simulink library "Contact_Forces_Lib"  (R2025b)
settings: Solver=ode45  StartTime=0.0  StopTime=10.0  RelTol=1e-3  EnableMultiTasking=on
undefined symbols (not defined in the file or in its folder): b_contact, custom_param_1, custom_param_2, Extr_Data_Ring, k_contact, l_cone, length_cylinder, length_tube, mu_kinetic, mu_static, pen_exponent, pen_full_damp_F, rad_s_cone, radius_cylinder, radius_tube, v_thr, X, Y, Z
libraries: nesl_utility x197, sm_lib x115, $bdroot x72, simulink x20, fl_lib x4
(part 11 of 12)

== system Contact_Forces_Lib/3D/Prototype/Cylinder In Ring Force/Point of Contact calc/Force Calc ==
  x : Inport
  y : Inport  Port=2
  v : Inport  Port=3
  z : Inport  Port=4
  th : Inport  Port=5
  Computing Force from nonzero penetration points : Subsystem  Commented=on
  Constant2 : Constant  Value=r_tube
  Dead Zone : DeadZone  LowerValue=-inf  UpperValue=0  ZeroCross=off
  MAX_ML : Subsystem  Commented=on
  MAX_SL : Subsystem
  Math Function : Math  Operator=square  SignedPower=on
  Math Function1 : Math  Operator=square  SignedPower=on
  Reciprocal Sqrt : Sqrt
  Sum : Sum  Inputs=|++
  Sum1 : Sum  Inputs=|+-
  Fx : Outport  VectorParamsAs1DForOutWhenUnconnected=off
  Fy : Outport  Port=2  VectorParamsAs1DForOutWhenUnconnected=off
  Fz : Outport  Port=3  VectorParamsAs1DForOutWhenUnconnected=off
  pc : Outport  Port=4  VectorParamsAs1DForOutWhenUnconnected=off
  maxpen : Outport  Port=5  VectorParamsAs1DForOutWhenUnconnected=off
  wires:
  y/1 -> MAX_SL/1(Y), Math Function1/1
  x/1 -> MAX_SL/2(X), Math Function/1
  Sum/1 -> Reciprocal Sqrt/1
  Reciprocal Sqrt/1 -> Sum1/1
  Constant2/1 -> Sum1/2
  Sum1/1 -> Dead Zone/1
  MAX_SL/1(Fx) -> Fx/1
  MAX_SL/2(Fy) -> Fy/1
  Dead Zone/1 -> MAX_SL/3(Pen)
  Math Function1/1 -> Sum/1
  Math Function/1 -> Sum/2
  v/1 -> MAX_SL/4(v)
  th/1 -> MAX_SL/5(th)
  z/1 -> MAX_SL/6(z)
  MAX_SL/4(pc) -> pc/1
  MAX_SL/3(Fz) -> Fz/1
  MAX_SL/5(maxpen) -> maxpen/1

== system Contact_Forces_Lib/3D/Prototype/Cylinder In Ring Force/Point of Contact calc/x calc ==
  note: Xb = r11*r*cos(th) + r12*r*sin(th) +r13*z + Xc;
  note: Find x coordinate in tube frame for cylinder point that is in the plane of the end of the tube
  r11 : Inport
  r12 : Inport  Port=2
  r13 : Inport  Port=3
  xc : Inport  Port=4
  th : Inport  Port=5
  z : Inport  Port=6
  Gain : Gain  Gain=r_cyl
  Gain1 : Gain  Gain=r_cyl
  Product : Product
  Product1 : Product
  Product2 : Product
  Sum : Sum  Inputs=|++++
  Trigonometric Function : Trigonometry  Operator=cos
  Trigonometric Function1 : Trigonometry
  x : Outport  VectorParamsAs1DForOutWhenUnconnected=off
  wires:
  th/1 -> Trigonometric Function/1, Trigonometric Function1/1
  Sum/1 -> x/1
  Product/1 -> Gain/1
  Gain1/1 -> Sum/3
  Trigonometric Function/1 -> Product/2
  Trigonometric Function1/1 -> Product1/2
  Gain/1 -> Sum/2
  Product1/1 -> Gain1/1
  r11/1 -> Product/1
  r12/1 -> Product1/1
  xc/1 -> Sum/1
  r13/1 -> Product2/1
  z/1 -> Product2/2
  Product2/1 -> Sum/4

== system Contact_Forces_Lib/3D/Prototype/Cylinder In Ring Force/Point of Contact calc/y calc ==
  note: Yb = r21*r*cos(th) + r22*r*sin(th) +r23*z + Yc;
  note: Find y coordinate in tube frame for cylinder point that is in the plane of the end of the tube
  r21 : Inport
  r22 : Inport  Port=2
  r23 : Inport  Port=3
  yc : Inport  Port=4
  th : Inport  Port=5
  z : Inport  Port=6
  Gain : Gain  Gain=r_cyl
  Gain1 : Gain  Gain=r_cyl
  Product : Product
  Product1 : Product
  Product2 : Product
  Sum : Sum  Inputs=|++++
  Trigonometric Function : Trigonometry  Operator=cos
  Trigonometric Function1 : Trigonometry
  y : Outport  VectorParamsAs1DForOutWhenUnconnected=off
  wires:
  Product2/1 -> Sum/4
  z/1 -> Product2/2
  r23/1 -> Product2/1
  yc/1 -> Sum/1
  r22/1 -> Product1/1
  r21/1 -> Product/1
  Product1/1 -> Gain1/1
  Gain/1 -> Sum/2
  Trigonometric Function1/1 -> Product1/2
  Trigonometric Function/1 -> Product/2
  Gain1/1 -> Sum/3
  Product/1 -> Gain/1
  Sum/1 -> y/1
  th/1 -> Trigonometric Function1/1, Trigonometric Function/1

== system Contact_Forces_Lib/3D/Prototype/Cylinder In Ring Force/Point of Contact calc/z calc ==
  note: Find z coordinate in cylinder frame for cylinder point that is in the plane of the end of the tube
  note: z = (L/2 - r31*r*cos(th) - r32*r*sin(th) - Zc)/r33;
  r31 : Inport
  r32 : Inport  Port=2
  r33 : Inport  Port=3
  zc : Inport  Port=4
  th : Inport  Port=5
  Constant : Constant  Value=l_tube/2
  Divide : Product  Inputs=*/
  Gain : Gain  Gain=r_cyl
  Gain1 : Gain  Gain=r_cyl
  Product : Product
  Product1 : Product
  Sum : Sum  Inputs=|---+
  Trigonometric Function : Trigonometry  Operator=cos
  Trigonometric Function1 : Trigonometry
  z : Outport  VectorParamsAs1DForOutWhenUnconnected=off
  wires:
  r32/1 -> Product1/1
  r31/1 -> Product/1
  Product1/1 -> Gain1/1
  Gain/1 -> Sum/2
  Trigonometric Function1/1 -> Product1/2
  Trigonometric Function/1 -> Product/2
  Gain1/1 -> Sum/3
  Product/1 -> Gain/1
  r33/1 -> Divide/2
  Constant/1 -> Sum/4
  Sum/1 -> Divide/1
  Divide/1 -> z/1
  zc/1 -> Sum/1
  th/1 -> Trigonometric Function1/1, Trigonometric Function/1

== system Contact_Forces_Lib/3D/Sphere in Sphere Force/Ff/Check w or v non zero/Else ==
  Action Port : ActionPort
  vabs_zero : Constant  Value=0  SampleTime=0
  vuvect_zero : Constant  Value=[0 0 0]  SampleTime=0
  vabs : Outport  InitialOutput=0  VectorParamsAs1DForOutWhenUnconnected=off
  vuvect : Outport  Port=2  InitialOutput=0  VectorParamsAs1DForOutWhenUnconnected=off
  wires:
  vabs_zero/1 -> vabs/1
  vuvect_zero/1 -> vuvect/1

== system Contact_Forces_Lib/3D/Sphere in Sphere Force/Ff/Check w or v non zero/mag v ==
  vect : Inport
  Add2 : Sum  Inputs=+++
  Demux : Demux  Outputs=3
  Math Function : Math  Operator=square  SignedPower=on
  Math Function1 : Math  Operator=square  SignedPower=on
  Math Function2 : Math  Operator=square  SignedPower=on
  Sqrt : Sqrt
  mag : Outport  VectorParamsAs1DForOutWhenUnconnected=off
  wires:
  Math Function2/1 -> Add2/3
  Demux/3 -> Math Function2/1
  Sqrt/1 -> mag/1
  Math Function1/1 -> Add2/2
  Math Function/1 -> Add2/1
  Add2/1 -> Sqrt/1
  vect/1 -> Demux/1
  Demux/1 -> Math Function/1
  Demux/2 -> Math Function1/1

== system Contact_Forces_Lib/3D/Sphere in Sphere Force/Ff/Check w or v non zero/mag w ==
  vect : Inport
  Add : Sum  Inputs=+++
  Demux : Demux  Outputs=3
  Math Function : Math  Operator=square  SignedPower=on
  Math Function1 : Math  Operator=square  SignedPower=on
  Math Function2 : Math  Operator=square  SignedPower=on
  Sqrt : Sqrt
  mag : Outport  VectorParamsAs1DForOutWhenUnconnected=off
  wires:
  Demux/2 -> Math Function1/1
  Demux/1 -> Math Function/1
  vect/1 -> Demux/1
  Add/1 -> Sqrt/1
  Math Function/1 -> Add/1
  Math Function1/1 -> Add/2
  Sqrt/1 -> mag/1
  Demux/3 -> Math Function2/1
  Math Function2/1 -> Add/3

== system Contact_Forces_Lib/3D/Sphere in Sphere Force/Ff/SlipVel/If Action Subsystem ==
  In1 : Inport
  In2 : Inport  Port=2
  Action Port : ActionPort
  Divide : Product  Inputs=/*
  Out1 : Outport  VectorParamsAs1DForOutWhenUnconnected=off
  wires:
  Divide/1 -> Out1/1
  In2/1 -> Divide/2
  In1/1 -> Divide/1

== system Contact_Forces_Lib/3D/Sphere in Sphere Force/Ff/SlipVel/mag ==
  vect : Inport
  Add2 : Sum  Inputs=+++
  Demux : Demux  Outputs=3
  Math Function : Math  Operator=square  SignedPower=on
  Math Function1 : Math  Operator=square  SignedPower=on
  Math Function2 : Math  Operator=square  SignedPower=on
  Sqrt : Sqrt
  mag : Outport  VectorParamsAs1DForOutWhenUnconnected=off
  wires:
  Math Function2/1 -> Add2/3
  Demux/3 -> Math Function2/1
  Sqrt/1 -> mag/1
  Math Function1/1 -> Add2/2
  Math Function/1 -> Add2/1
  Add2/1 -> Sqrt/1
  vect/1 -> Demux/1
  Demux/1 -> Math Function/1
  Demux/2 -> Math Function1/1

== system Contact_Forces_Lib/3D/Sphere to Cone Force/Forces/Ff/Relative vel at CP ==
  note: Calculate relative velocity at contact point between sphere and tube. Two components: about ring and along tube axis. Use magnitude to calculate friction force, atan2 retains relative magnitude and direction between the components.
  InOut : Inport
  rad : Inport  Port=2
  vrad : Inport  Port=3
  Pen : Inport  Port=4
  vazm : Inport  Port=5
  vazmx : Inport  Port=6
  vazmy : Inport  Port=7
  wzf : Inport  Port=8
  vzf : Inport  Port=9
  wxf : Inport  Port=10
  wyf : Inport  Port=11
  azm : Inport  Port=12
  Calculate vRelFace : Subsystem
  Calculate vRelRing : Subsystem
  Follower Radius : Constant  Value=radius_sphere
  Math Function : Math  Operator=square  SignedPower=on
  Math Function1 : Math  Operator=square  SignedPower=on
  Midpt Pen : Gain  Gain=0.5
  Product1 : Product
  Sqrt : Sqrt
  Sum1 : Sum  Inputs=+-
  Sum3 : Sum  Inputs=|++
  Trigonometric Function : Trigonometry  Operator=atan2
  vRelAbs : Outport  VectorParamsAs1DForOutWhenUnconnected=off
  rSphtoCP : Outport  Port=2  VectorParamsAs1DForOutWhenUnconnected=off
  rConAxtoCP : Outport  Port=3  VectorParamsAs1DForOutWhenUnconnected=off
  alpha : Outport  Port=4  VectorParamsAs1DForOutWhenUnconnected=off
  wires:
  vrad/1 -> Calculate vRelFace/6(vrad)
  vazmy/1 -> Calculate vRelRing/6(vazmy)
  vazmx/1 -> Calculate vRelRing/5(vazmx)
  Product1/1 -> Calculate vRelRing/1(rSphtoCP sign), Calculate vRelFace/1(rSphtoCP sign)
  Sum1/1 -> Product1/1, rSphtoCP/1  "rSphtoCP"
  InOut/1 -> Product1/2  "InOut"
  Trigonometric Function/1 -> alpha/1  "alpha"
  Sqrt/1 -> vRelAbs/1
  Sum3/1 -> Sqrt/1
  Math Function/1 -> Sum3/1
  Math Function1/1 -> Sum3/2
  Follower Radius/1 -> Sum1/1
  Pen/1 -> Midpt Pen/1
  Midpt Pen/1 -> Sum1/2
  Calculate vRelFace/1(vRelFace) -> Math Function1/1, Trigonometric Function/1  "vRelFace"
  wxf/1 -> Calculate vRelFace/3(wxf), Calculate vRelRing/8(wxf)
  vzf/1 -> Calculate vRelFace/5(vzf)
  azm/1 -> Calculate vRelFace/2(azm), Calculate vRelRing/7(azm)
  wyf/1 -> Calculate vRelRing/9(wyf), Calculate vRelFace/4(wyf)
  Calculate vRelRing/2(vRelRing) -> Math Function/1, Trigonometric Function/2  "vRelRing"
  rad/1 -> Calculate vRelRing/2(rad)
  vazm/1 -> Calculate vRelRing/3(vazm)
  wzf/1 -> Calculate vRelRing/4(wzf)
  Calculate vRelRing/1(rConAxtoCP) -> rConAxtoCP/1

== system Contact_Forces_Lib/3D/Sphere to Cone Force/Forces/Ff/Resolve Ff ==
  note: Resolve Friction Force in
      | Sphere F reference frame
  note: Resolve Friction Force in
      | Cone B reference frame
  InOut : Inport
  Ff : Inport  Port=2
  R : Inport  Port=3
  z : Inport  Port=4
  rSphtoCP : Inport  Port=5
  rConAxtoCP : Inport  Port=6
  alpha : Inport  Port=7
  azm : Inport  Port=8
  Ff in ConB : Subsystem
  Ff in SphF : Subsystem
  FxSphF : Outport  VectorParamsAs1DForOutWhenUnconnected=off
  FySphF : Outport  Port=2  VectorParamsAs1DForOutWhenUnconnected=off
  FzSphF : Outport  Port=3  VectorParamsAs1DForOutWhenUnconnected=off
  TSphF : Outport  Port=4  VectorParamsAs1DForOutWhenUnconnected=off
  FxConB : Outport  Port=5  VectorParamsAs1DForOutWhenUnconnected=off
  FyConB : Outport  Port=6  VectorParamsAs1DForOutWhenUnconnected=off
  FzConB : Outport  Port=7  VectorParamsAs1DForOutWhenUnconnected=off
  TConB : Outport  Port=8  VectorParamsAs1DForOutWhenUnconnected=off
  wires:
  Ff in SphF/4(TSphF) -> TSphF/1
  Ff in ConB/4(TSphF_B) -> Ff in SphF/4(TSphF_B)
  Ff in ConB/5(TConB) -> TConB/1
  alpha/1 -> Ff in ConB/4(alpha)
  Ff in ConB/3(FzConB) -> FzConB/1, Ff in SphF/3(FzConB)
  Ff in SphF/3(FzSphF) -> FzSphF/1
  R/1 -> Ff in SphF/5(R)
  azm/1 -> Ff in ConB/3(azm)
  Ff in SphF/2(FxSphF) -> FxSphF/1
  Ff in ConB/2(FyConB) -> Ff in SphF/2(FyConB), FyConB/1
  Ff in ConB/1(FxConB) -> FxConB/1, Ff in SphF/1(FxConB)
  Ff in SphF/1(FySphF) -> FySphF/1
  Ff/1 -> Ff in ConB/2(Ff)
  rConAxtoCP/1 -> Ff in ConB/6(rConAxtoCP)
  rSphtoCP/1 -> Ff in ConB/5(rSphtoCP)
  z/1 -> Ff in ConB/7(z)
  InOut/1 -> Ff in ConB/1(InOut)

== system Contact_Forces_Lib/3D/Sphere to Cone Force/Forces/Fn/Equiv Torques ==
  azm : Inport
  FxConB : Inport  Port=2
  FyConB : Inport  Port=3
  FzConB : Inport  Port=4
  rad : Inport  Port=5
  z : Inport  Port=6
  Constant : Constant  Value=radius_sphere*sinConeTh
  Constant1 : Constant  Value=radius_sphere*cosConeTh
  Product : Product  Inputs=3
  Product1 : Product
  Product2 : Product  Inputs=3
  Product3 : Product
  Sum : Sum
  Sum1 : Sum  Inputs=+-
  Sum2 : Sum
  Sum3 : Sum  Inputs=+-
  sin : Trigonometry
  sin1 : Trigonometry  Operator=cos
  TxConB : Outport  VectorParamsAs1DForOutWhenUnconnected=off
  TyConB : Outport  Port=2  VectorParamsAs1DForOutWhenUnconnected=off
  wires:
  sin1/1 -> Product2/2
  sin/1 -> Product/2
  Sum/1 -> Product/3, Product2/3
  Sum3/1 -> TyConB/1
  Sum1/1 -> TxConB/1
  rad/1 -> Sum/1
  Product3/1 -> Sum3/1
  Product/1 -> Sum1/1
  Constant1/1 -> Sum2/2
  Sum2/1 -> Product3/2, Product1/2
  Constant/1 -> Sum/2
  z/1 -> Sum2/1
  Product1/1 -> Sum1/2
  Product2/1 -> Sum3/2
  azm/1 -> sin/1, sin1/1
  FxConB/1 -> Product3/1
  FzConB/1 -> Product/1, Product2/1
  FyConB/1 -> Product1/1

== system Contact_Forces_Lib/3D/Sphere to Cone Force/Forces/Fn/Fn in SphF ==
  R : Inport
  FxConB : Inport  Port=2
  FyConB : Inport  Port=3
  FzConB : Inport  Port=4
  Demux : Demux  Outputs=3
  Divide3 : Product  Inputs=/*  Multiplication=Matrix(*)
  Gain : Gain  Gain=-1
  Mux1 : Mux  Inputs=3
  FySphF : Outport  VectorParamsAs1DForOutWhenUnconnected=off
  FxSphF : Outport  Port=2  VectorParamsAs1DForOutWhenUnconnected=off
  FzSphF : Outport  Port=3  VectorParamsAs1DForOutWhenUnconnected=off
  wires:
  FzConB/1 -> Mux1/3
  Gain/1 -> Demux/1
  R/1 -> Divide3/1
  Demux/1 -> FxSphF/1
  Demux/2 -> FySphF/1
  Demux/3 -> FzSphF/1
  FxConB/1 -> Mux1/1
  FyConB/1 -> Mux1/2
  Mux1/1 -> Divide3/2
  Divide3/1 -> Gain/1

== system Contact_Forces_Lib/3D/Sphere to Cone Force/Forces/Fn/Fn in TubB ==
  Fn : Inport
  azm : Inport  Port=2
  Divide1 : Product  Inputs=**
  Divide2 : Product  Inputs=**
  Gain : Gain  Gain=sinConeTh
  Gain1 : Gain  Gain=sinConeTh
  cos : Trigonometry  Operator=cos
  sin : Trigonometry
  FxConB : Outport  VectorParamsAs1DForOutWhenUnconnected=off
  FyConB : Outport  Port=2  VectorParamsAs1DForOutWhenUnconnected=off
  FzConB : Outport  Port=3  VectorParamsAs1DForOutWhenUnconnected=off
  wires:
  Gain1/1 -> FzConB/1
  Gain/1 -> Divide1/1, Divide2/1
  Fn/1 -> Gain/1, Gain1/1
  azm/1 -> cos/1, sin/1
  sin/1 -> Divide2/2
  cos/1 -> Divide1/2
  Divide1/1 -> FxConB/1
  Divide2/1 -> FyConB/1

== system Contact_Forces_Lib/3D/Sphere to Cone Force/Sensing/rad_azm_cal/rad_0 ==
  Action Port : ActionPort
  Zeros : Constant  Value=[0 0 0 0]  SampleTime=0
  F : Outport  InitialOutput=[0]  VectorParamsAs1DForOutWhenUnconnected=off
  wires:
  Zeros/1 -> F/1

== system Contact_Forces_Lib/3D/Sphere to Cone Force/Sensing/rad_azm_cal/rad_azm_cal ==
  note: vazm = (x*vy - y*vx)/(x^2+y^2)
  note: vrad = (x*vx + y*vy)/z
  note: azm = atan2(y, x)
  note: rad = sqrt(x^2+y^2)
  x : Inport
  y : Inport  Port=2
  vx : Inport  Port=3
  vy : Inport  Port=4
  Action Port : ActionPort
  Add : Sum
  Add1 : Sum  Inputs=+-
  Divide : Product  Inputs=*/
  Divide1 : Product  Inputs=*/
  Math Function : Math  Operator=square  SignedPower=on
  Math Function1 : Math  Operator=square  SignedPower=on
  Mux : Mux
  Product{,1..3} (4 alike) : Product
  Sqrt : Sqrt
  Sum : Sum
  Trigonometric Function : Trigonometry  Operator=atan2
  F : Outport  VectorParamsAs1DForOutWhenUnconnected=off
  wires:
  Math Function1/1 -> Sum/2
  Math Function/1 -> Sum/1
  Sum/1 -> Divide1/2, Sqrt/1
  Trigonometric Function/1 -> Mux/2  "azm"
  x/1 -> Trigonometric Function/2, Product/1, Product2/1, Math Function/1
  y/1 -> Trigonometric Function/1, Product1/1, Product3/1, Math Function1/1
  vx/1 -> Product3/2, Product/2
  vy/1 -> Product2/2, Product1/2
  Product/1 -> Add/1
  Product1/1 -> Add/2
  Add/1 -> Divide/1
  Sqrt/1 -> Mux/1, Divide/2  "rad"
  Divide/1 -> Mux/3  "vrad"
  Product2/1 -> Add1/1
  Product3/1 -> Add1/2
  Add1/1 -> Divide1/1
  Divide1/1 -> Mux/4  "vazm"
  Mux/1 -> F/1

== system Contact_Forces_Lib/3D/Sphere to Cone Force/Sensing/rad_azm_cal/vazmx_0 ==
  Action Port : ActionPort
  Zeros : Constant  Value=0  SampleTime=0
  F : Outport  InitialOutput=[0]  VectorParamsAs1DForOutWhenUnconnected=off
  wires:
  Zeros/1 -> F/1

== system Contact_Forces_Lib/3D/Sphere to Cone Force/Sensing/rad_azm_cal/vazmx_cal ==
  note: vazmx = (y*vz - z*vy)/(y^2+z^2)
  y : Inport
  z : Inport  Port=2
  vy : Inport  Port=3
  vz : Inport  Port=4
  Action Port : ActionPort
  Add2 : Sum  Inputs=+-
  Divide2 : Product  Inputs=*/
  Math Function1 : Math  Operator=square  SignedPower=on
  Math Function2 : Math  Operator=square  SignedPower=on
  Product4 : Product
  Product5 : Product
  Sum1 : Sum
  vazmx : Outport  VectorParamsAs1DForOutWhenUnconnected=off
  wires:
  Product4/1 -> Add2/1
  Product5/1 -> Add2/2
  Add2/1 -> Divide2/1
  vy/1 -> Product5/2
  y/1 -> Math Function1/1, Product4/1
  Math Function1/1 -> Sum1/1
  z/1 -> Product5/1, Math Function2/1
  Math Function2/1 -> Sum1/2
  Sum1/1 -> Divide2/2
  vz/1 -> Product4/2
  Divide2/1 -> vazmx/1  "vazmx"

== system Contact_Forces_Lib/3D/Sphere to Cone Force/Sensing/rad_azm_cal/vazmy_0 ==
  Action Port : ActionPort
  Zeros : Constant  Value=0  SampleTime=0
  F : Outport  InitialOutput=[0]  VectorParamsAs1DForOutWhenUnconnected=off
  wires:
  Zeros/1 -> F/1

== system Contact_Forces_Lib/3D/Sphere to Cone Force/Sensing/rad_azm_cal/vazmy_cal ==
  note: vazmy = (z*vx - x*vz)/(z^2+x^2)
  x : Inport
  z : Inport  Port=2
  vx : Inport  Port=3
  vz : Inport  Port=4
  Action Port : ActionPort
  Add3 : Sum  Inputs=+-
  Divide3 : Product  Inputs=*/
  Math Function : Math  Operator=square  SignedPower=on
  Math Function2 : Math  Operator=square  SignedPower=on
  Product6 : Product
  Product7 : Product
  Sum2 : Sum
  vazmy : Outport  VectorParamsAs1DForOutWhenUnconnected=off
  wires:
  vx/1 -> Product6/2
  x/1 -> Math Function/1, Product7/1
  Math Function/1 -> Sum2/1
  Add3/1 -> Divide3/1
  Product7/1 -> Add3/2
  Product6/1 -> Add3/1
  z/1 -> Product6/1, Math Function2/1
  Math Function2/1 -> Sum2/2
  Sum2/1 -> Divide3/2
  vz/1 -> Product7/2
  Divide3/1 -> vazmy/1  "vazmy"

== system Contact_Forces_Lib/3D/Sphere to Plane Force/Forces/Ff/SlipVel ==
  wx : Inport
  wy : Inport  Port=2
  vx : Inport  Port=3
  vy : Inport  Port=4
  Fx1 : Constant  Value=sphere_rad
  Math Function : Math  Operator=square  SignedPower=on
  Math Function1 : Math  Operator=square  SignedPower=on
  Product3 : Product
  Product4 : Product
  Sqrt : Sqrt
  Sum1 : Sum  Inputs=|++
  Sum2 : Sum  Inputs=|-+
  Sum3 : Sum  Inputs=|++
  Trigonometric Function : Trigonometry  Operator=atan2
  vabs : Outport  VectorParamsAs1DForOutWhenUnconnected=off
  alpha : Outport  Port=2  VectorParamsAs1DForOutWhenUnconnected=off
  wires:
  Sum2/1 -> Math Function1/1, Trigonometric Function/2  "slipx"
  Sum1/1 -> Math Function/1, Trigonometric Function/1  "slipy"
  Math Function1/1 -> Sum3/2
  Math Function/1 -> Sum3/1
  Sum3/1 -> Sqrt/1
  Sqrt/1 -> vabs/1
  Trigonometric Function/1 -> alpha/1
  Product4/1 -> Sum2/1
  vy/1 -> Sum1/2
  Fx1/1 -> Product4/1, Product3/2
  vx/1 -> Sum2/2
  wy/1 -> Product4/2
  Product3/1 -> Sum1/1
  wx/1 -> Product3/1

== system Contact_Forces_Lib/3D/Sphere to Plane Force Enabled/Forces/Ff/SlipVel ==
  wx : Inport
  wy : Inport  Port=2
  vx : Inport  Port=3
  vy : Inport  Port=4
  Fx1 : Constant  Value=sphere_rad
  Math Function : Math  Operator=square  SignedPower=on
  Math Function1 : Math  Operator=square  SignedPower=on
  Product3 : Product
  Product4 : Product
  Sqrt : Sqrt
  Sum1 : Sum  Inputs=|++
  Sum2 : Sum  Inputs=|-+
  Sum3 : Sum  Inputs=|++
  Trigonometric Function : Trigonometry  Operator=atan2
  vabs : Outport  VectorParamsAs1DForOutWhenUnconnected=off
  alpha : Outport  Port=2  VectorParamsAs1DForOutWhenUnconnected=off
  wires:
  wx/1 -> Product3/1
  Product3/1 -> Sum1/1
  wy/1 -> Product4/2
  vx/1 -> Sum2/2
  Fx1/1 -> Product3/2, Product4/1
  vy/1 -> Sum1/2
  Product4/1 -> Sum2/1
  Trigonometric Function/1 -> alpha/1
  Sqrt/1 -> vabs/1
  Sum3/1 -> Sqrt/1
  Math Function/1 -> Sum3/1
  Math Function1/1 -> Sum3/2
  Sum1/1 -> Trigonometric Function/1, Math Function/1  "slipy"
  Sum2/1 -> Trigonometric Function/2, Math Function1/1  "slipx"

== system Contact_Forces_Lib/3D/Sphere to Sphere Force/Ff/Check w or v non zero/Else ==
  Action Port : ActionPort
  Constant : Constant  Value=0  SampleTime=0
  Constant1 : Constant  Value=[0 0 0]  SampleTime=0
  vabs : Outport  InitialOutput=0  VectorParamsAs1DForOutWhenUnconnected=off
  vuvect : Outport  Port=2  InitialOutput=0  VectorParamsAs1DForOutWhenUnconnected=off
  wires:
  Constant1/1 -> vuvect/1
  Constant/1 -> vabs/1

== system Contact_Forces_Lib/3D/Sphere to Sphere Force/Ff/Check w or v non zero/mag v ==
  vect : Inport
  Add2 : Sum  Inputs=+++
  Demux : Demux  Outputs=3
  Math Function : Math  Operator=square  SignedPower=on
  Math Function1 : Math  Operator=square  SignedPower=on
  Math Function2 : Math  Operator=square  SignedPower=on
  Sqrt : Sqrt
  mag : Outport  VectorParamsAs1DForOutWhenUnconnected=off
  wires:
  Demux/2 -> Math Function1/1
  Demux/1 -> Math Function/1
  vect/1 -> Demux/1
  Add2/1 -> Sqrt/1
  Math Function/1 -> Add2/1
  Math Function1/1 -> Add2/2
  Sqrt/1 -> mag/1
  Demux/3 -> Math Function2/1
  Math Function2/1 -> Add2/3

== system Contact_Forces_Lib/3D/Sphere to Sphere Force/Ff/Check w or v non zero/mag w ==
  vect : Inport
  Add : Sum  Inputs=+++
  Demux : Demux  Outputs=3
  Math Function : Math  Operator=square  SignedPower=on
  Math Function1 : Math  Operator=square  SignedPower=on
  Math Function2 : Math  Operator=square  SignedPower=on
  Sqrt : Sqrt
  mag : Outport  VectorParamsAs1DForOutWhenUnconnected=off
  wires:
  Math Function2/1 -> Add/3
  Demux/3 -> Math Function2/1
  Sqrt/1 -> mag/1
  Math Function1/1 -> Add/2
  Math Function/1 -> Add/1
  Add/1 -> Sqrt/1
  vect/1 -> Demux/1
  Demux/1 -> Math Function/1
  Demux/2 -> Math Function1/1

== system Contact_Forces_Lib/3D/Sphere to Sphere Force/Ff/SlipVel/If Action Subsystem ==
  In1 : Inport
  In2 : Inport  Port=2
  Action Port : ActionPort
  Divide : Product  Inputs=/*
  Out1 : Outport  VectorParamsAs1DForOutWhenUnconnected=off
  wires:
  In1/1 -> Divide/1
  In2/1 -> Divide/2
  Divide/1 -> Out1/1

== system Contact_Forces_Lib/3D/Sphere to Sphere Force/Ff/SlipVel/mag ==
  vect : Inport
  Add2 : Sum  Inputs=+++
  Demux : Demux  Outputs=3
  Math Function : Math  Operator=square  SignedPower=on
  Math Function1 : Math  Operator=square  SignedPower=on
  Math Function2 : Math  Operator=square  SignedPower=on
  Sqrt : Sqrt
  mag : Outport  VectorParamsAs1DForOutWhenUnconnected=off
  wires:
  Demux/2 -> Math Function1/1
  Demux/1 -> Math Function/1
  vect/1 -> Demux/1
  Add2/1 -> Sqrt/1
  Math Function/1 -> Add2/1
  Math Function1/1 -> Add2/2
  Sqrt/1 -> mag/1
  Demux/3 -> Math Function2/1
  Math Function2/1 -> Add2/3

== system Contact_Forces_Lib/3D/Sphere to Tube Force/Forces/Ff/Relative vel at CP ==
  note: Calculate relative velocity at contact point between sphere and tube. Two components: about ring and along tube axis. Use magnitude to calculate friction force, atan2 retains relative magnitude and direction between the components.
  Fn : Inport
  rad : Inport  Port=2
  Pen : Inport  Port=3
  vazm : Inport  Port=4
  wzf : Inport  Port=5
  vzf : Inport  Port=6
  wxf : Inport  Port=7
  wyf : Inport  Port=8
  azm : Inport  Port=9
  Calculate vRelAxis : Subsystem
  Calculate vRelRing : Subsystem
  Follower Radius : Constant  Value=radius_sphere
  Math Function : Math  Operator=square  SignedPower=on
  Math Function1 : Math  Operator=square  SignedPower=on
  Midpt Pen : Gain  Gain=0.5
  Product1 : Product
  Sign : Signum  ZeroCross=off
  Sqrt : Sqrt
  Sum1 : Sum  Inputs=+-
  Sum3 : Sum  Inputs=|++
  Trigonometric Function : Trigonometry  Operator=atan2
  vRelAbs : Outport  VectorParamsAs1DForOutWhenUnconnected=off
  rSphtoCP : Outport  Port=2  VectorParamsAs1DForOutWhenUnconnected=off
  rCyltoCP : Outport  Port=3  VectorParamsAs1DForOutWhenUnconnected=off
  alpha : Outport  Port=4  VectorParamsAs1DForOutWhenUnconnected=off
  wires:
  Calculate vRelRing/1(rCyltoCP) -> rCyltoCP/1
  wzf/1 -> Calculate vRelRing/3(wzf)
  vazm/1 -> Calculate vRelRing/2(vazm)
  rad/1 -> Calculate vRelRing/1(rad)
  Calculate vRelRing/2(vRelRing) -> Math Function/1, Trigonometric Function/2  "vRelRing"
  wyf/1 -> Calculate vRelAxis/5(wyf)
  azm/1 -> Calculate vRelAxis/4(azm)
  vzf/1 -> Calculate vRelAxis/3(vzf)
  wxf/1 -> Calculate vRelAxis/2(wxf)
  Calculate vRelAxis/1(vRelAxis) -> Trigonometric Function/1, Math Function1/1  "vRelAxis"
  Midpt Pen/1 -> Sum1/2
  Fn/1 -> Sign/1
  Pen/1 -> Midpt Pen/1
  Follower Radius/1 -> Sum1/1
  Math Function1/1 -> Sum3/2
  Math Function/1 -> Sum3/1
  Sum3/1 -> Sqrt/1
  Sqrt/1 -> vRelAbs/1
  Trigonometric Function/1 -> alpha/1  "alpha"
  Sign/1 -> Product1/2  "InOut"
  Sum1/1 -> Product1/1, rSphtoCP/1  "rSphtoCP"
  Product1/1 -> Calculate vRelAxis/1(rSphtoCP sign), Calculate vRelRing/4(rSphtoCP sign)

== system Contact_Forces_Lib/3D/Sphere to Tube Force/Forces/Ff/Resolve Ff ==
  note: Resolve Friction Force in
      | Tube B reference frame
  note: Resolve Friction Force in
      | Sphere F reference frame
  InOut : Inport
  Ff : Inport  Port=2
  rSphtoCP : Inport  Port=3
  rCyltoCP : Inport  Port=4
  alpha : Inport  Port=5
  z : Inport  Port=6
  R : Inport  Port=7
  azm : Inport  Port=8
  Ff in SphF : Subsystem
  Ff in TubB : Subsystem
  FxSphF : Outport  VectorParamsAs1DForOutWhenUnconnected=off
  FySphF : Outport  Port=2  VectorParamsAs1DForOutWhenUnconnected=off
  FzSphF : Outport  Port=3  VectorParamsAs1DForOutWhenUnconnected=off
  TSphF : Outport  Port=4  VectorParamsAs1DForOutWhenUnconnected=off
  FxSphB : Outport  Port=5  VectorParamsAs1DForOutWhenUnconnected=off
  FyTubB : Outport  Port=6  VectorParamsAs1DForOutWhenUnconnected=off
  FzTubB : Outport  Port=7  VectorParamsAs1DForOutWhenUnconnected=off
  TTubB : Outport  Port=8  VectorParamsAs1DForOutWhenUnconnected=off
  wires:
  InOut/1 -> Ff in TubB/1(InOut)
  z/1 -> Ff in TubB/7(z)
  rSphtoCP/1 -> Ff in TubB/5(rSphtoCP)
  rCyltoCP/1 -> Ff in TubB/6(rCyltoCP)
  Ff/1 -> Ff in TubB/2(Ff)
  Ff in SphF/1(FySphF) -> FySphF/1
  Ff in TubB/1(FxTubB) -> Ff in SphF/1(FxTubB), FxSphB/1
  Ff in TubB/2(FyTubB) -> FyTubB/1, Ff in SphF/2(FyTubB)
  Ff in SphF/2(FxSphF) -> FxSphF/1
  azm/1 -> Ff in TubB/3(azm)
  R/1 -> Ff in SphF/5(R)
  Ff in SphF/3(FzSphF) -> FzSphF/1
  Ff in TubB/3(FzTubB) -> Ff in SphF/3(FzTubB), FzTubB/1
  alpha/1 -> Ff in TubB/4(alpha)
  Ff in TubB/5(TTubB) -> TTubB/1
  Ff in TubB/4(TSphF_B) -> Ff in SphF/4(TSphF_B)
  Ff in SphF/4(TSphF) -> TSphF/1

== system Contact_Forces_Lib/3D/Sphere to Tube Force/Forces/Fn/Fn in SphF ==
  R : Inport
  FxTubB : Inport  Port=2
  FyTubB : Inport  Port=3
  Constant : Constant  Value=0
  Demux : Demux  Outputs=3
  Divide3 : Product  Inputs=/*  Multiplication=Matrix(*)
  Gain : Gain  Gain=-1
  Mux1 : Mux  Inputs=3
  FySphF : Outport  VectorParamsAs1DForOutWhenUnconnected=off
  FxSphF : Outport  Port=2  VectorParamsAs1DForOutWhenUnconnected=off
  FzSphF : Outport  Port=3  VectorParamsAs1DForOutWhenUnconnected=off
  wires:
  Divide3/1 -> Gain/1
  Mux1/1 -> Divide3/2
  FyTubB/1 -> Mux1/2
  FxTubB/1 -> Mux1/1
  Demux/3 -> FzSphF/1
  Demux/2 -> FySphF/1
  Demux/1 -> FxSphF/1
  Constant/1 -> Mux1/3
  R/1 -> Divide3/1
  Gain/1 -> Demux/1

== system Contact_Forces_Lib/3D/Sphere to Tube Force/Forces/Fn/Fn in TubB ==
  Fn : Inport
  azm : Inport  Port=2
  Divide1 : Product  Inputs=**
  Divide2 : Product  Inputs=**
  cos : Trigonometry  Operator=cos
  sin : Trigonometry
  FxTubB : Outport  VectorParamsAs1DForOutWhenUnconnected=off
  FyTubB : Outport  Port=2  VectorParamsAs1DForOutWhenUnconnected=off
  wires:
  Divide2/1 -> FyTubB/1
  Divide1/1 -> FxTubB/1
  cos/1 -> Divide1/2
  sin/1 -> Divide2/2
  azm/1 -> sin/1, cos/1
  Fn/1 -> Divide2/1, Divide1/1

== system Contact_Forces_Lib/3D/Sphere to Tube Force/Sensing/rad_azm_cal/rad_0 ==
  Action Port : ActionPort
  Zeros : Constant  Value=[0 0 0 0]  SampleTime=0
  F : Outport  InitialOutput=[0]  VectorParamsAs1DForOutWhenUnconnected=off
  wires:
  Zeros/1 -> F/1

== system Contact_Forces_Lib/3D/Sphere to Tube Force/Sensing/rad_azm_cal/rad_azm_cal ==
  note: z = sqrt(x2+y2)
      | zdot = 1/z(x*xdot+y*ydot)
      | azm = atan(y/x)
      | azmdot = 1/z2(x*ydot-xdot*y)
  X : Inport
  Y : Inport  Port=2
  Xdot : Inport  Port=3
  Ydot : Inport  Port=4
  Action Port : ActionPort
  Add : Sum
  Add1 : Sum  Inputs=+-
  Divide : Product  Inputs=*/
  Divide1 : Product  Inputs=*/
  Math Function : Math  Operator=square  SignedPower=on
  Math Function1 : Math  Operator=square  SignedPower=on
  Mux : Mux
  Product{,1..3} (4 alike) : Product
  Sqrt : Sqrt
  Sum : Sum  Inputs=|++
  Trigonometric Function : Trigonometry  Operator=atan2
  F : Outport  VectorParamsAs1DForOutWhenUnconnected=off
  wires:
  Mux/1 -> F/1
  Divide1/1 -> Mux/4
  Add1/1 -> Divide1/1
  Product3/1 -> Add1/2
  Product2/1 -> Add1/1
  Divide/1 -> Mux/3
  Sqrt/1 -> Divide/2, Mux/1
  Add/1 -> Divide/1
  Product1/1 -> Add/2
  Product/1 -> Add/1
  Ydot/1 -> Product1/2, Product2/2
  Xdot/1 -> Product/2, Product3/2
  Y/1 -> Math Function1/1, Product1/1, Product3/1, Trigonometric Function/1
  X/1 -> Math Function/1, Product/1, Product2/1, Trigonometric Function/2
  Trigonometric Function/1 -> Mux/2
  Sum/1 -> Sqrt/1, Divide1/2
  Math Function/1 -> Sum/1
  Math Function1/1 -> Sum/2

== system Contact_Forces_Lib/3D/Sphere to Tube Force Enabled/Forces/Ff/Relative vel at CP ==
  note: Calculate relative velocity at contact point between sphere and tube. Two components: about ring and along tube axis. Use magnitude to calculate friction force, atan2 retains relative magnitude and direction between the components.
  Fn : Inport
  rad : Inport  Port=2
  Pen : Inport  Port=3
  vazm : Inport  Port=4
  wzf : Inport  Port=5
  vzf : Inport  Port=6
  wxf : Inport  Port=7
  wyf : Inport  Port=8
  azm : Inport  Port=9
  Calculate vRelAxis : Subsystem
  Calculate vRelRing : Subsystem
  Follower Radius : Constant  Value=radius_sphere
  Math Function : Math  Operator=square  SignedPower=on
  Math Function1 : Math  Operator=square  SignedPower=on
  Midpt Pen : Gain  Gain=0.5
  Product1 : Product
  Sign : Signum  ZeroCross=off
  Sqrt : Sqrt
  Sum1 : Sum  Inputs=+-
  Sum3 : Sum  Inputs=|++
  Trigonometric Function : Trigonometry  Operator=atan2
  vRelAbs : Outport  VectorParamsAs1DForOutWhenUnconnected=off
  rSphtoCP : Outport  Port=2  VectorParamsAs1DForOutWhenUnconnected=off
  rCyltoCP : Outport  Port=3  VectorParamsAs1DForOutWhenUnconnected=off
  alpha : Outport  Port=4  VectorParamsAs1DForOutWhenUnconnected=off
  wires:
  Calculate vRelRing/1(rCyltoCP) -> rCyltoCP/1
  wzf/1 -> Calculate vRelRing/3(wzf)
  vazm/1 -> Calculate vRelRing/2(vazm)
  rad/1 -> Calculate vRelRing/1(rad)
  Calculate vRelRing/2(vRelRing) -> Math Function/1, Trigonometric Function/2  "vRelRing"
  wyf/1 -> Calculate vRelAxis/5(wyf)
  azm/1 -> Calculate vRelAxis/4(azm)
  vzf/1 -> Calculate vRelAxis/3(vzf)
  wxf/1 -> Calculate vRelAxis/2(wxf)
  Calculate vRelAxis/1(vRelAxis) -> Trigonometric Function/1, Math Function1/1  "vRelAxis"
  Midpt Pen/1 -> Sum1/2
  Fn/1 -> Sign/1
  Pen/1 -> Midpt Pen/1
  Follower Radius/1 -> Sum1/1
  Math Function1/1 -> Sum3/2
  Math Function/1 -> Sum3/1
  Sum3/1 -> Sqrt/1
  Sqrt/1 -> vRelAbs/1
  Trigonometric Function/1 -> alpha/1  "alpha"
  Sign/1 -> Product1/2  "InOut"
  Sum1/1 -> Product1/1, rSphtoCP/1  "rSphtoCP"
  Product1/1 -> Calculate vRelAxis/1(rSphtoCP sign), Calculate vRelRing/4(rSphtoCP sign)

== system Contact_Forces_Lib/3D/Sphere to Tube Force Enabled/Forces/Ff/Resolve Ff ==
  note: Resolve Friction Force in
      | Tube B reference frame
  note: Resolve Friction Force in
      | Sphere F reference frame
  InOut : Inport
  Ff : Inport  Port=2
  rSphtoCP : Inport  Port=3
  rCyltoCP : Inport  Port=4
  alpha : Inport  Port=5
  z : Inport  Port=6
  R : Inport  Port=7
  azm : Inport  Port=8
  Ff in SphF : Subsystem
  Ff in TubB : Subsystem
  FxSphF : Outport  VectorParamsAs1DForOutWhenUnconnected=off
  FySphF : Outport  Port=2  VectorParamsAs1DForOutWhenUnconnected=off
  FzSphF : Outport  Port=3  VectorParamsAs1DForOutWhenUnconnected=off
  TSphF : Outport  Port=4  VectorParamsAs1DForOutWhenUnconnected=off
  FxSphB : Outport  Port=5  VectorParamsAs1DForOutWhenUnconnected=off
  FyTubB : Outport  Port=6  VectorParamsAs1DForOutWhenUnconnected=off
  FzTubB : Outport  Port=7  VectorParamsAs1DForOutWhenUnconnected=off
  TTubB : Outport  Port=8  VectorParamsAs1DForOutWhenUnconnected=off
  wires:
  InOut/1 -> Ff in TubB/1(InOut)
  z/1 -> Ff in TubB/7(z)
  rSphtoCP/1 -> Ff in TubB/5(rSphtoCP)
  rCyltoCP/1 -> Ff in TubB/6(rCyltoCP)
  Ff/1 -> Ff in TubB/2(Ff)
  Ff in SphF/1(FySphF) -> FySphF/1
  Ff in TubB/1(FxTubB) -> Ff in SphF/1(FxTubB), FxSphB/1
  Ff in TubB/2(FyTubB) -> FyTubB/1, Ff in SphF/2(FyTubB)
  Ff in SphF/2(FxSphF) -> FxSphF/1
  azm/1 -> Ff in TubB/3(azm)
  R/1 -> Ff in SphF/5(R)
  Ff in SphF/3(FzSphF) -> FzSphF/1
  Ff in TubB/3(FzTubB) -> Ff in SphF/3(FzTubB), FzTubB/1
  alpha/1 -> Ff in TubB/4(alpha)
  Ff in TubB/5(TTubB) -> TTubB/1
  Ff in TubB/4(TSphF_B) -> Ff in SphF/4(TSphF_B)
  Ff in SphF/4(TSphF) -> TSphF/1

== system Contact_Forces_Lib/3D/Sphere to Tube Force Enabled/Forces/Fn/Fn in SphF ==
  R : Inport
  FxTubB : Inport  Port=2
  FyTubB : Inport  Port=3
  Constant : Constant  Value=0
  Demux : Demux  Outputs=3
  Divide3 : Product  Inputs=/*  Multiplication=Matrix(*)
  Gain : Gain  Gain=-1
  Mux1 : Mux  Inputs=3
  FySphF : Outport  VectorParamsAs1DForOutWhenUnconnected=off
  FxSphF : Outport  Port=2  VectorParamsAs1DForOutWhenUnconnected=off
  FzSphF : Outport  Port=3  VectorParamsAs1DForOutWhenUnconnected=off
  wires:
  Divide3/1 -> Gain/1
  Mux1/1 -> Divide3/2
  FyTubB/1 -> Mux1/2
  FxTubB/1 -> Mux1/1
  Demux/3 -> FzSphF/1
  Demux/2 -> FySphF/1
  Demux/1 -> FxSphF/1
  Constant/1 -> Mux1/3
  R/1 -> Divide3/1
  Gain/1 -> Demux/1

== system Contact_Forces_Lib/3D/Sphere to Tube Force Enabled/Forces/Fn/Fn in TubB ==
  Fn : Inport
  azm : Inport  Port=2
  Divide1 : Product  Inputs=**
  Divide2 : Product  Inputs=**
  cos : Trigonometry  Operator=cos
  sin : Trigonometry
  FxTubB : Outport  VectorParamsAs1DForOutWhenUnconnected=off
  FyTubB : Outport  Port=2  VectorParamsAs1DForOutWhenUnconnected=off
  wires:
  Divide2/1 -> FyTubB/1
  Divide1/1 -> FxTubB/1
  cos/1 -> Divide1/2
  sin/1 -> Divide2/2
  azm/1 -> sin/1, cos/1
  Fn/1 -> Divide2/1, Divide1/1

== system Contact_Forces_Lib/3D/Sphere to Tube Force Enabled/Sensing/rad_azm_cal/rad_0 ==
  Action Port : ActionPort
  Zeros : Constant  Value=[0 0 0 0]  SampleTime=0
  F : Outport  InitialOutput=[0]  VectorParamsAs1DForOutWhenUnconnected=off
  wires:
  Zeros/1 -> F/1

== system Contact_Forces_Lib/3D/Sphere to Tube Force Enabled/Sensing/rad_azm_cal/rad_azm_cal ==
  note: z = sqrt(x2+y2)
      | zdot = 1/z(x*xdot+y*ydot)
      | azm = atan(y/x)
      | azmdot = 1/z2(x*ydot-xdot*y)
  X : Inport
  Y : Inport  Port=2
  Xdot : Inport  Port=3
  Ydot : Inport  Port=4
  Action Port : ActionPort
  Add : Sum
  Add1 : Sum  Inputs=+-
  Divide : Product  Inputs=*/
  Divide1 : Product  Inputs=*/
  Math Function : Math  Operator=square  SignedPower=on
  Math Function1 : Math  Operator=square  SignedPower=on
  Mux : Mux
  Product{,1..3} (4 alike) : Product
  Sqrt : Sqrt
  Sum : Sum  Inputs=|++
  Trigonometric Function : Trigonometry  Operator=atan2
  F : Outport  VectorParamsAs1DForOutWhenUnconnected=off
  wires:
  Mux/1 -> F/1
  Divide1/1 -> Mux/4
  Add1/1 -> Divide1/1
  Product3/1 -> Add1/2
  Product2/1 -> Add1/1
  Divide/1 -> Mux/3
  Sqrt/1 -> Divide/2, Mux/1
  Add/1 -> Divide/1
  Product1/1 -> Add/2
  Product/1 -> Add/1
  Ydot/1 -> Product1/2, Product2/2
  Xdot/1 -> Product/2, Product3/2
  Y/1 -> Math Function1/1, Product1/1, Product3/1, Trigonometric Function/1
  X/1 -> Math Function/1, Product/1, Product2/1, Trigonometric Function/2
  Trigonometric Function/1 -> Mux/2
  Sum/1 -> Sqrt/1, Divide1/2
  Math Function/1 -> Sum/1
  Math Function1/1 -> Sum/2

== system Contact_Forces_Lib/2D/Circle to Finite Line Force/Forces/Resolve Forces/Friction/VCirPt ==
  wz : Inport
  X sep : Inport  Port=2
  Constant : Constant  Value=line_depth
  Product : Product
  Product1 : Product
  Sign1 : Signum
  Subtract : Sum  Inputs=+-
  vCir : Outport  VectorParamsAs1DForOutWhenUnconnected=off
  wires:
  wz/1 -> Product1/1
  Product1/1 -> vCir/1
  Product/1 -> Subtract/2
  Sign1/1 -> Product/1
  X sep/1 -> Subtract/1, Sign1/1
  Constant/1 -> Product/2
  Subtract/1 -> Product1/2

== system Contact_Forces_Lib/2D/Circle to Finite Line Force Enabled/Forces/Resolve Forces/Friction/VCirPt ==
  wz : Inport
  X sep : Inport  Port=2
  Constant : Constant  Value=line_depth
  Product : Product
  Product1 : Product
  Sign1 : Signum
  Subtract : Sum  Inputs=+-
  vCir : Outport  VectorParamsAs1DForOutWhenUnconnected=off
  wires:
  Subtract/1 -> Product1/2
  Constant/1 -> Product/2
  X sep/1 -> Sign1/1, Subtract/1
  Sign1/1 -> Product/1
  Product/1 -> Subtract/2
  Product1/1 -> vCir/1
  wz/1 -> Product1/1

== system Contact_Forces_Lib/2D/Circle to Ring Force/Forces/Ff/Resolve Ff/Ff in CirB ==
  Ff : Inport
  azm : Inport  Port=2
  Divide1 : Product  Inputs=**
  Divide2 : Product  Inputs=**
  Gain1 : Gain
  Gain3 : Gain  Gain=-1
  cos : Trigonometry
  deg2rad : Gain  Gain=pi/180
  sin : Trigonometry  Operator=cos
  FxRinB : Outport  VectorParamsAs1DForOutWhenUnconnected=off
  FyRinB : Outport  Port=2  VectorParamsAs1DForOutWhenUnconnected=off
  wires:
  Gain1/1 -> Divide2/1, Divide1/1
  azm/1 -> deg2rad/1
  Divide2/1 -> FyRinB/1
  cos/1 -> Gain3/1
  sin/1 -> Divide2/2
  deg2rad/1 -> sin/1, cos/1
  Divide1/1 -> FxRinB/1
  Ff/1 -> Gain1/1
  Gain3/1 -> Divide1/2

== system Contact_Forces_Lib/2D/Circle to Ring Force/Forces/Ff/Resolve Ff/Ff in CirF ==
  R : Inport
  FxRinB : Inport  Port=2
  FyRinB : Inport  Port=3
  Demux : Demux  Outputs=2
  Divide3 : Product  Inputs=**  Multiplication=Matrix(*)
  Gain1 : Gain  Gain=-1
  Mux1 : Mux  Inputs=2
  FyCirF : Outport  VectorParamsAs1DForOutWhenUnconnected=off
  FxCirF : Outport  Port=2  VectorParamsAs1DForOutWhenUnconnected=off
  wires:
  R/1 -> Divide3/1
  Divide3/1 -> Gain1/1
  Mux1/1 -> Divide3/2
  Gain1/1 -> Demux/1
  Demux/1 -> FyCirF/1
  Demux/2 -> FxCirF/1
  FyRinB/1 -> Mux1/1
  FxRinB/1 -> Mux1/2

== system Contact_Forces_Lib/2D/Circle to Ring Force/Forces/Ff/Resolve Ff/Tz ==
  rCirFtoCP : Inport
  rRinBtoCP : Inport  Port=2
  Ff : Inport  Port=3
  Divide4 : Product  Inputs=**
  Divide5 : Product  Inputs=**
  Gain2 : Gain  Gain=-1
  TzRinB : Outport  VectorParamsAs1DForOutWhenUnconnected=off
  TzCirF : Outport  Port=2  VectorParamsAs1DForOutWhenUnconnected=off
  wires:
  rRinBtoCP/1 -> Divide5/2
  Divide5/1 -> TzRinB/1
  rCirFtoCP/1 -> Divide4/2
  Divide4/1 -> TzCirF/1
  Gain2/1 -> Divide5/1
  Ff/1 -> Divide4/1, Gain2/1

== system Contact_Forces_Lib/3D/Prototype/Cone in Ring Force/Point of Contact calc/Force Calc/Computing Force from nonzero penetration points ==
  Y : Inport
  X : Inport  Port=2
  Pen : Inport  Port=3
  Derivative : Derivative  Commented=on  CoefficientInTFapproximation=1e-4
  For Each Subsystem1 : Subsystem  Commented=on  TreatAsAtomicUnit=on
  For Iterator Subsystem : Subsystem  Commented=on  TreatAsAtomicUnit=on
  Gain1 : Gain  Commented=on  Gain=-1
  Linear1 : Subsystem  Commented=on  VariantControl=Linear  mask(Linear Force Law){k_pen=1e4, b_penvel=1e3}
      mask prompts: k_pen "Contact Stiffness"; b_penvel "Contact Damping"
      mask help: Implements a contact force law as a linear spring damper. The damping force is applied only as the penetration depth increases.
      mask Help: web(which('Force_Laws.html'));
  Product2 : Product  Commented=on
  Product3 : Product  Commented=on
  Sum of Elements : Sum  Commented=on  Inputs=+
  Sum of Elements1 : Sum  Commented=on  Inputs=+
  Sum3 : Sum  Commented=on  Inputs=|+-
  Trigonometric Function3 : Trigonometry  Commented=on  Operator=atan2
  Trigonometric Function4 : Trigonometry  Commented=on  Operator=cos
  Trigonometric Function5 : Trigonometry  Commented=on
  Fx : Outport  VectorParamsAs1DForOutWhenUnconnected=off
  Fy : Outport  Port=2  VectorParamsAs1DForOutWhenUnconnected=off
  wires:
  Trigonometric Function3/1 -> Trigonometric Function5/1, Trigonometric Function4/1
  Linear1/2(Damp F) -> Sum3/2
  Trigonometric Function5/1 -> Product3/1
  Trigonometric Function4/1 -> Product2/1
  Gain1/1 -> Product2/2, Product3/2
  Sum3/1 -> Gain1/1
  Linear1/1(Spr F) -> Sum3/1
  Sum of Elements1/1 -> Fy/1
  Pen/1 -> Derivative/1, For Each Subsystem1/1(In1), Linear1/1(Pen)
  X/1 -> Trigonometric Function3/2
  Y/1 -> Trigonometric Function3/1
  Sum of Elements/1 -> Fx/1
  Derivative/1 -> Linear1/2(Pen Vel)
  Product2/1 -> Sum of Elements/1
  Product3/1 -> Sum of Elements1/1

== system Contact_Forces_Lib/3D/Prototype/Cone in Ring Force/Point of Contact calc/Force Calc/MAX_ML ==
  Y : Inport
  X : Inport  Port=2
  pen : Inport  Port=3
  Gain : Gain  Gain=-1
  Linear : Subsystem  VariantControl=Linear  mask(Linear Force Law){k_pen=k_stiff, b_penvel=b_damp}
      mask prompts: k_pen "Contact Stiffness"; b_penvel "Contact Damping"
      mask help: Implements a contact force law as a linear spring damper. The damping force is applied only as the penetration depth increases.
      mask Help: web(which('Force_Laws.html'));
  MATLAB Function : MATLAB Function  TreatAsAtomicUnit=on
  Product : Product
  Product1 : Product
  Sum2 : Sum  Inputs=|+-
  Transfer Fcn : TransferFcn  Numerator=[1 0]  Denominator=[1e-4 1]
  Trigonometric Function : Trigonometry  Operator=atan2
  Trigonometric Function1 : Trigonometry  Operator=cos
  Trigonometric Function2 : Trigonometry
  Fx : Outport  VectorParamsAs1DForOutWhenUnconnected=off
  Fy : Outport  Port=2  VectorParamsAs1DForOutWhenUnconnected=off
  wires:
  Product1/1 -> Fy/1
  MATLAB Function/4(ind) -> ?
  X/1 -> MATLAB Function/2(x)
  Product/1 -> Fx/1
  pen/1 -> MATLAB Function/1(pen)
  Transfer Fcn/1 -> Linear/2(Pen Vel)
  Gain/1 -> Product1/2, Product/2
  Trigonometric Function1/1 -> Product/1
  Linear/1(Spr F) -> Sum2/1
  Trigonometric Function2/1 -> Product1/1
  Sum2/1 -> Gain/1
  Linear/2(Damp F) -> Sum2/2
  Trigonometric Function/1 -> Trigonometric Function1/1, Trigonometric Function2/1
  Y/1 -> MATLAB Function/3(y)
  MATLAB Function/2(yc) -> Trigonometric Function/1
  MATLAB Function/1(xc) -> Trigonometric Function/2
  MATLAB Function/3(penc) -> Transfer Fcn/1, Linear/1(Pen)

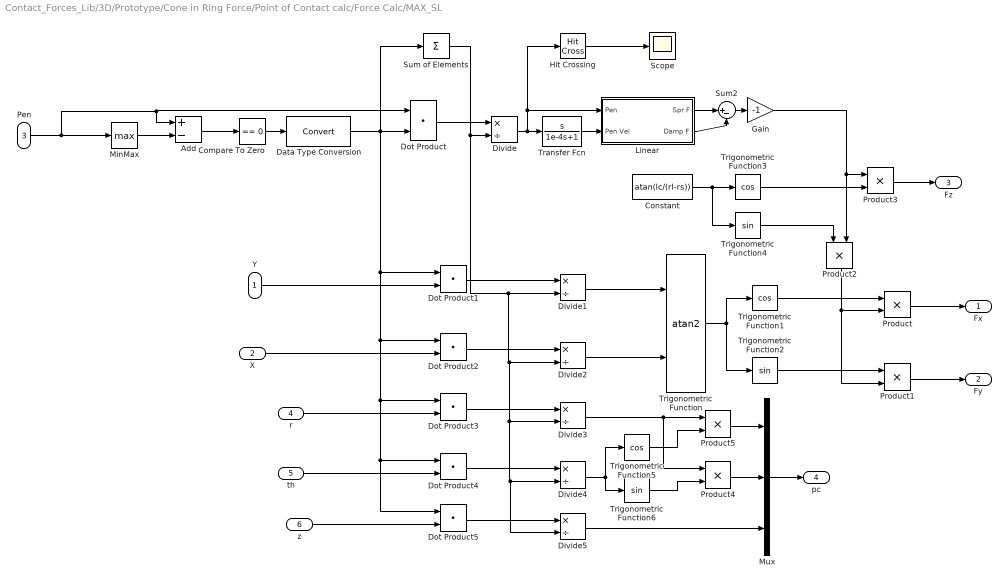
== system Contact_Forces_Lib/3D/Prototype/Cone in Ring Force/Point of Contact calc/Force Calc/MAX_SL ==
  Y : Inport
  X : Inport  Port=2
  Pen : Inport  Port=3
  r : Inport  Port=4
  th : Inport  Port=5
  z : Inport  Port=6
  Add : Sum  Inputs=+-
  Compare To Zero : simulink/Logic and Bit Operations/Compare To Zero  relop===  OutDataTypeStr=boolean  ZeroCross=off
  Constant : Constant  Value=atan(lc/(rl-rs))
  Data Type Conversion : DataTypeConversion  SaturateOnIntegerOverflow=off  RndMeth=Floor
  Divide{,1..5} (6 alike) : Product  Inputs=*/
  Dot Product{,1..5} (6 alike) : DotProduct  OutDataTypeStr=Inherit: Inherit via internal rule
  Gain : Gain  Gain=-1
  Hit Crossing : HitCross
  Linear : Subsystem  VariantControl=Linear  mask(Linear Force Law){k_pen=k_stiff, b_penvel=b_damp}
      mask prompts: k_pen "Contact Stiffness"; b_penvel "Contact Damping"
      mask help: Implements a contact force law as a linear spring damper. The damping force is applied only as the penetration depth increases.
      mask Help: web(which('Force_Laws.html'));
  MinMax : MinMax  Function=max  ZeroCross=off
  Mux : Mux  Inputs=3
  Product{,1..5} (6 alike) : Product
  Scope : Scope
      settings: DataLoggingVariableName=ScopeData2  DataLoggingSaveFormat=Array
  Sum of Elements : Sum  Inputs=+
  Sum2 : Sum  Inputs=|+-
  Transfer Fcn : TransferFcn  Numerator=[1 0]  Denominator=[1e-4 1]
  Trigonometric Function : Trigonometry  Operator=atan2
  Trigonometric Function1 : Trigonometry  Operator=cos
  Trigonometric Function2 : Trigonometry
  Trigonometric Function3 : Trigonometry  Operator=cos
  Trigonometric Function4 : Trigonometry
  Trigonometric Function5 : Trigonometry  Operator=cos
  Trigonometric Function6 : Trigonometry
  Fx : Outport  VectorParamsAs1DForOutWhenUnconnected=off
  Fy : Outport  Port=2  VectorParamsAs1DForOutWhenUnconnected=off
  Fz : Outport  Port=3  VectorParamsAs1DForOutWhenUnconnected=off
  pc : Outport  Port=4  VectorParamsAs1DForOutWhenUnconnected=off
  wires:
  Trigonometric Function/1 -> Trigonometric Function2/1, Trigonometric Function1/1
  Linear/2(Damp F) -> Sum2/2
  Sum2/1 -> Gain/1
  Trigonometric Function2/1 -> Product1/1
  Linear/1(Spr F) -> Sum2/1
  Trigonometric Function1/1 -> Product/1
  Transfer Fcn/1 -> Linear/2(Pen Vel)
  MinMax/1 -> Add/2
  Add/1 -> Compare To Zero/1
  Compare To Zero/1 -> Data Type Conversion/1
  Product/1 -> Fx/1
  Pen/1 -> Dot Product/1, Add/1, MinMax/1
  Product1/1 -> Fy/1
  Y/1 -> Dot Product1/2
  X/1 -> Dot Product2/2
  Data Type Conversion/1 -> Dot Product/2, Dot Product1/1, Dot Product5/1, Dot Product4/1, Dot Product3/1, Dot Product2/1, Sum of Elements/1
  Dot Product/1 -> Divide/1
  Sum of Elements/1 -> Divide1/2, Divide5/2, Divide4/2, Divide3/2, Divide2/2, Divide/2
  Dot Product1/1 -> Divide1/1
  Dot Product2/1 -> Divide2/1
  Divide1/1 -> Trigonometric Function/1
  Divide2/1 -> Trigonometric Function/2
  Divide/1 -> Hit Crossing/1, Linear/1(Pen), Transfer Fcn/1
  Hit Crossing/1 -> Scope/1
  Constant/1 -> Trigonometric Function4/1, Trigonometric Function3/1
  Trigonometric Function4/1 -> Product2/1
  Gain/1 -> Product3/1, Product2/2
  Product2/1 -> Product1/2, Product/2
  Product3/1 -> Fz/1
  Trigonometric Function3/1 -> Product3/2
  Mux/1 -> pc/1
  Dot Product3/1 -> Divide3/1
  Dot Product4/1 -> Divide4/1
  Dot Product5/1 -> Divide5/1
  r/1 -> Dot Product3/2
  th/1 -> Dot Product4/2
  z/1 -> Dot Product5/2
  Divide5/1 -> Mux/3
  Product4/1 -> Mux/2
  Product5/1 -> Mux/1
  Divide4/1 -> Trigonometric Function5/1, Trigonometric Function6/1
  Divide3/1 -> Product4/1, Product5/1
  Trigonometric Function5/1 -> Product5/2
  Trigonometric Function6/1 -> Product4/2

== system Contact_Forces_Lib/3D/Prototype/Cylinder In Ring Force/Point of Contact calc/Force Calc/Computing Force from nonzero penetration points ==
  Y : Inport
  X : Inport  Port=2
  Pen : Inport  Port=3
  Derivative : Derivative  Commented=on  CoefficientInTFapproximation=1e-4
  For Each Subsystem1 : Subsystem  Commented=on  TreatAsAtomicUnit=on
  For Iterator Subsystem : Subsystem  Commented=on  TreatAsAtomicUnit=on
  Gain1 : Gain  Commented=on  Gain=-1
  Linear1 : Subsystem  Commented=on  VariantControl=Linear  mask(Linear Force Law){k_pen=1e4, b_penvel=1e3}
      mask prompts: k_pen "Contact Stiffness"; b_penvel "Contact Damping"
      mask help: Implements a contact force law as a linear spring damper. The damping force is applied only as the penetration depth increases.
      mask Help: web(which('Force_Laws.html'));
  Product2 : Product  Commented=on
  Product3 : Product  Commented=on
  Sum of Elements : Sum  Commented=on  Inputs=+
  Sum of Elements1 : Sum  Commented=on  Inputs=+
  Sum3 : Sum  Commented=on  Inputs=|+-
  Trigonometric Function3 : Trigonometry  Commented=on  Operator=atan2
  Trigonometric Function4 : Trigonometry  Commented=on  Operator=cos
  Trigonometric Function5 : Trigonometry  Commented=on
  Fx : Outport  VectorParamsAs1DForOutWhenUnconnected=off
  Fy : Outport  Port=2  VectorParamsAs1DForOutWhenUnconnected=off
  wires:
  Trigonometric Function3/1 -> Trigonometric Function5/1, Trigonometric Function4/1
  Linear1/2(Damp F) -> Sum3/2
  Trigonometric Function5/1 -> Product3/1
  Trigonometric Function4/1 -> Product2/1
  Gain1/1 -> Product2/2, Product3/2
  Sum3/1 -> Gain1/1
  Linear1/1(Spr F) -> Sum3/1
  Sum of Elements1/1 -> Fy/1
  Pen/1 -> Derivative/1, For Each Subsystem1/1(In1), Linear1/1(Pen)
  X/1 -> Trigonometric Function3/2
  Y/1 -> Trigonometric Function3/1
  Sum of Elements/1 -> Fx/1
  Derivative/1 -> Linear1/2(Pen Vel)
  Product2/1 -> Sum of Elements/1
  Product3/1 -> Sum of Elements1/1

== system Contact_Forces_Lib/3D/Prototype/Cylinder In Ring Force/Point of Contact calc/Force Calc/MAX_ML ==
  Y : Inport
  X : Inport  Port=2
  pen : Inport  Port=3
  Gain : Gain  Gain=-1
  Linear : Subsystem  VariantControl=Linear  mask(Linear Force Law){k_pen=1e5, b_penvel=1e3}
      mask prompts: k_pen "Contact Stiffness"; b_penvel "Contact Damping"
      mask help: Implements a contact force law as a linear spring damper. The damping force is applied only as the penetration depth increases.
      mask Help: web(which('Force_Laws.html'));
  MATLAB Function : MATLAB Function  TreatAsAtomicUnit=on
  Product : Product
  Product1 : Product
  Sum2 : Sum  Inputs=|+-
  Transfer Fcn : TransferFcn  Numerator=[1 0]  Denominator=[1e-4 1]
  Trigonometric Function : Trigonometry  Operator=atan2
  Trigonometric Function1 : Trigonometry  Operator=cos
  Trigonometric Function2 : Trigonometry
  Fx : Outport  VectorParamsAs1DForOutWhenUnconnected=off
  Fy : Outport  Port=2  VectorParamsAs1DForOutWhenUnconnected=off
  wires:
  Product1/1 -> Fy/1
  MATLAB Function/4(ind) -> ?
  X/1 -> MATLAB Function/2(x)
  Product/1 -> Fx/1
  pen/1 -> MATLAB Function/1(pen)
  Transfer Fcn/1 -> Linear/2(Pen Vel)
  Gain/1 -> Product1/2, Product/2
  Trigonometric Function1/1 -> Product/1
  Linear/1(Spr F) -> Sum2/1
  Trigonometric Function2/1 -> Product1/1
  Sum2/1 -> Gain/1
  Linear/2(Damp F) -> Sum2/2
  Trigonometric Function/1 -> Trigonometric Function1/1, Trigonometric Function2/1
  Y/1 -> MATLAB Function/3(y)
  MATLAB Function/2(yc) -> Trigonometric Function/1
  MATLAB Function/1(xc) -> Trigonometric Function/2
  MATLAB Function/3(penc) -> Transfer Fcn/1, Linear/1(Pen)
